simulink model "WBR_Simulator"  (R2023b)
settings: Solver=FixedStepAuto  StartTime=0.0  StopTime=60  FixedStep=0.001  MaxStep=0.001
undefined symbols (not defined in the file or in its folder): DiscIntNeverNeededParam, magnitude, robot_stats, SIMPARAM, X, Y, Z
libraries: sm_lib x73, nesl_utility x50, simulink x17, slpidlib x6, dsparch4 x2
(part 7 of 7)

== system WBR_Simulator/腿建模/并联腿1/运动学解算验证(仅可证明旋转矩阵 ==
  R : Inport
  R_inv : Inport  Port=2
  Bus Creator1 : BusCreator  Inputs=2
  Bus Creator3 : BusCreator  Inputs=2
  Discrete Derivative : simulink/Discrete/Discrete Derivative  gainval=1.0  ICPrevScaledInput=0.0  OutMin=[]  OutMax=[]  OutDataType=fixdt(1, 16)  OutScaling=2^-10  DoSatur=off
  Discrete Derivative1 : simulink/Discrete/Discrete Derivative  gainval=1.0  ICPrevScaledInput=0.0  OutMin=[]  OutMax=[]  OutDataType=fixdt(1, 16)  OutScaling=2^-10  DoSatur=off
  Mux : Mux  Inputs=2
  Mux1 : Mux  Inputs=2
  PS-Simulink Converter{4..7} (4 alike) : nesl_utility/PS-Simulink Converter  PhysicalDomain=network_engine_domain  SubClassName=ps_output  LeftPortType=input  RightPortType=output  PseudoPeriodic=off  Frequencies=[]  VectorFormat=1-D array  Unit=inherit  AffineConversion=off
  Product : Product
  Product1 : Product  Multiplication=Matrix(*)
  Product2 : Product  Multiplication=Matrix(*)
  Transform Sensor : sm_lib/Frames and Transforms/Transform Sensor  MeasurementFrame=Base  RotationSequence=XYX  SenseAngle=off  SenseAxis=off  SenseQ=off  SenseR=off  SenseRotationSequence=off  SenseOmegaX=off  SenseOmegaY=off  SenseOmegaZ=off  SenseOmega=off  SenseQDot=off  SenseRDot=off  SenseRotationSequenceDot=off  SenseAlphaX=off  SenseAlphaY=off  SenseAlphaZ=off  SenseAlpha=off  SenseQDDot=off  SenseRDDot=off  SenseX=on  SenseY=off  SenseZ=on  SenseXYZ=off  SenseRad=off  SenseAzim=off  SenseDist=off  SenseInc=off  SenseXDot=on  SenseYDot=off  SenseZDot=on  SenseXYZDot=off  SenseRadDot=off  SenseAzimDot=off  SenseDistDot=off  SenseIncDot=off  SenseXDDot=off  SenseYDDot=off  SenseZDDot=off  SenseXYZDDot=off  SenseRadDDot=off  SenseAzimDDot=off  SenseDistDDot=off  SenseIncDDot=off
  Zero-Order Hold{,1..3} (4 alike) : ZeroOrderHold  SampleTime=0.001
  笛卡尔转极坐标 : Subsystem
  五连杆末端坐标 : PMIOPort  Side=Right
  基坐标 : PMIOPort  Port=2  Side=Left
  wires:
  Discrete Derivative/1 -> Product/1
  Product1/1 -> ?  "代算C点正交坐标速度"
  [R] -> Product2/1
  Discrete Derivative1/1 -> Mux/2, Bus Creator1/2  "vd"
  笛卡尔转极坐标/2(L_0) -> Discrete Derivative1/1, Product/2
  Mux/1 -> Product1/2
  笛卡尔转极坐标/1(phi_0) -> Discrete Derivative/1
  [R_inv] -> Product1/1
  Product/1 -> Mux/1, Bus Creator1/1  "vq"
  PS-Simulink Converter5/1 -> Zero-Order Hold1/1
  Bus Creator1/1 -> ?  "真实C点极坐标速度"
  PS-Simulink Converter4/1 -> Zero-Order Hold/1
  Mux1/1 -> Product2/2
  Product2/1 -> ?  "代算C点极坐标速度"
  Bus Creator3/1 -> ?  "真实C点正交坐标速度"
  R/1 -> [R]
  R_inv/1 -> [R_inv]
  Zero-Order Hold/1 -> 笛卡尔转极坐标/1(x)
  Zero-Order Hold1/1 -> 笛卡尔转极坐标/2(z)
  Zero-Order Hold3/1 -> Mux1/2, Bus Creator3/2
  PS-Simulink Converter7/1 -> Zero-Order Hold3/1  "vz"
  Zero-Order Hold2/1 -> Mux1/1, Bus Creator3/1
  PS-Simulink Converter6/1 -> Zero-Order Hold2/1  "vx"
  connections:
  PS-Simulink Converter5/LConn1 -- Transform Sensor/RConn3
  PS-Simulink Converter4/LConn1 -- Transform Sensor/RConn2
  Transform Sensor/RConn1 -- 五连杆末端坐标/RConn1
  基坐标/RConn1 -- Transform Sensor/LConn1
  PS-Simulink Converter6/LConn1 -- Transform Sensor/RConn4
  PS-Simulink Converter7/LConn1 -- Transform Sensor/RConn5

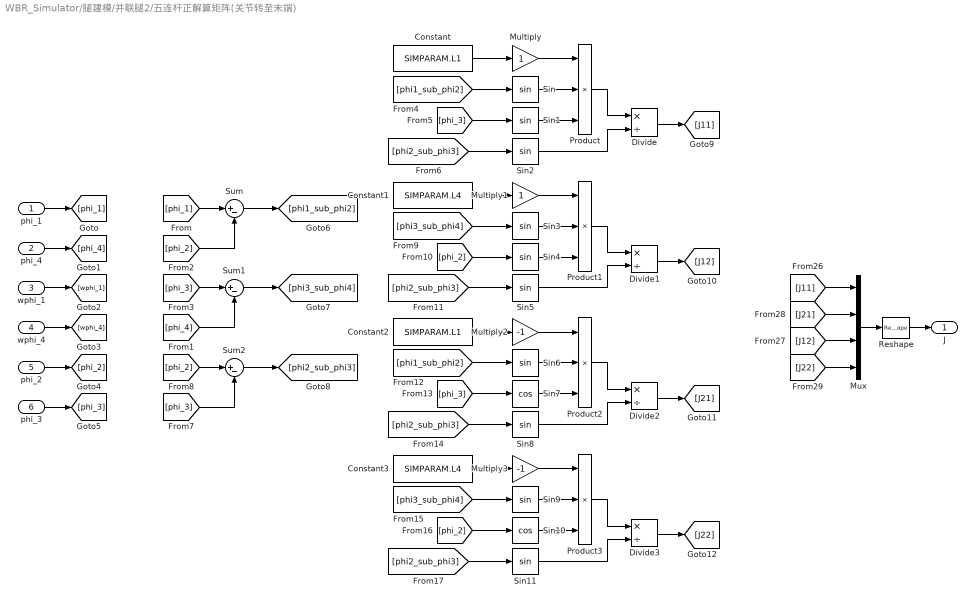
== system WBR_Simulator/腿建模/并联腿2/五连杆正解算矩阵(关节转至末端) ==
  phi_1 : Inport
  phi_4 : Inport  Port=2
  wphi_1 : Inport  Port=3
  wphi_4 : Inport  Port=4
  phi_2 : Inport  Port=5
  phi_3 : Inport  Port=6
  Constant : Constant  Value=SIMPARAM.L1
  Constant1 : Constant  Value=SIMPARAM.L4
  Constant2 : Constant  Value=SIMPARAM.L1
  Constant3 : Constant  Value=SIMPARAM.L4
  Divide{,1..3} (4 alike) : Product  Inputs=*/
  Multiply : Gain
  Multiply1 : Gain
  Multiply2 : Gain  Gain=-1
  Multiply3 : Gain  Gain=-1
  Mux : Mux
  Product{,1..3} (4 alike) : Product  Inputs=3
  Reshape : Reshape  OutputDimensionality=Customize  OutputDimensions=[2,2]
  Sin{,1..6,8..9,11} (10 alike) : Trigonometry
  Sin10 : Trigonometry  Operator=cos
  Sin7 : Trigonometry  Operator=cos
  Sum : Sum  Inputs=|+-
  Sum1 : Sum  Inputs=|+-
  Sum2 : Sum  Inputs=|+-
  J : Outport
  wires:
  phi_1/1 -> [phi_1]
  phi_4/1 -> [phi_4]
  wphi_1/1 -> [wphi_1]
  wphi_4/1 -> [wphi_4]
  phi_2/1 -> [phi_2]
  phi_3/1 -> [phi_3]
  [phi_1] -> Sum/1
  [phi_2] -> Sum/2
  Sum/1 -> [phi1_sub_phi2]
  Sum1/1 -> [phi3_sub_phi4]
  [phi_3] -> Sum1/1
  [phi_4] -> Sum1/2
  [phi1_sub_phi2] -> Sin/1
  Sin/1 -> Product/2
  Constant/1 -> Multiply/1
  Multiply/1 -> Product/1
  [phi_3] -> Sin1/1
  Sin1/1 -> Product/3
  Product/1 -> Divide/1
  [phi2_sub_phi3] -> Sin2/1
  Sin2/1 -> Divide/2
  [phi_3] -> Sum2/2
  [phi_2] -> Sum2/1
  Sum2/1 -> [phi2_sub_phi3]
  Divide/1 -> [J11]
  Product1/1 -> Divide1/1
  Constant1/1 -> Multiply1/1
  [phi3_sub_phi4] -> Sin3/1
  Divide1/1 -> [J12]
  Sin5/1 -> Divide1/2
  [phi_2] -> Sin4/1
  Multiply1/1 -> Product1/1
  Sin4/1 -> Product1/3
  [phi2_sub_phi3] -> Sin5/1
  Sin3/1 -> Product1/2
  Product2/1 -> Divide2/1
  Constant2/1 -> Multiply2/1
  [phi1_sub_phi2] -> Sin6/1
  Divide2/1 -> [J21]
  Sin8/1 -> Divide2/2
  [phi_3] -> Sin7/1
  Multiply2/1 -> Product2/1
  Sin7/1 -> Product2/3
  [phi2_sub_phi3] -> Sin8/1
  Sin6/1 -> Product2/2
  Product3/1 -> Divide3/1
  Constant3/1 -> Multiply3/1
  [phi3_sub_phi4] -> Sin9/1
  Divide3/1 -> [J22]
  Sin11/1 -> Divide3/2
  [phi_2] -> Sin10/1
  Multiply3/1 -> Product3/1
  Sin10/1 -> Product3/3
  [phi2_sub_phi3] -> Sin11/1
  Sin9/1 -> Product3/2
  [J11] -> Mux/1
  [J22] -> Mux/4
  Mux/1 -> Reshape/1
  Reshape/1 -> J/1
  [J21] -> Mux/2
  [J12] -> Mux/3

== system WBR_Simulator/腿建模/并联腿2/腿末端控制器 ==
  phi : Inport
  wphi_1 : Inport  Port=2
  wphi_4 : Inport  Port=3
  set_tq : Inport  Port=4
  set_fd : Inport  Port=5
  J : Inport  Port=6
  Bus Selector : BusSelector  OutputSignals=phi_1,phi_2
  Constant : Constant  Value=0
  Constant1 : Constant
  Constant2 : Constant
  Constant3 : Constant  Value=0
  Divide : Product  Inputs=*/
  Mux : Mux  Inputs=2
  Mux1 : Mux
  Product : Product  Inputs=/  Multiplication=Matrix(*)
  Product8 : Product  Multiplication=Matrix(*)
  Reshape : Reshape  OutputDimensionality=Customize  OutputDimensions=[2,2]
  极坐标运动控制器 : Subsystem
  笛卡尔坐标系转极坐标系 : Subsystem
  torque_1 : Outport
  torque_4 : Outport  Port=2
  R : Outport  Port=3
  R_inv : Outport  Port=4
  phi_0 : Outport  Port=5
  L_0 : Outport  Port=6
  real_vq : Outport  Port=7
  real_vd : Outport  Port=8
  valid_tqd : Outport  Port=9
  wires:
  J/1 -> [J]
  wphi_1/1 -> [wphi_1]
  wphi_4/1 -> [wphi_4]
  Product8/1 -> [real_vxy]
  [wphi_4] -> Mux/2
  [J] -> Product8/1
  Mux/1 -> Product8/2
  [wphi_1] -> Mux/1
  [real_vxy] -> 极坐标运动控制器/1(real_vxy)
  [R] -> 极坐标运动控制器/2(R)
  [J] -> 极坐标运动控制器/3(J)
  笛卡尔坐标系转极坐标系/1(R) -> [R], R/1, Product/1
  Product/1 -> R_inv/1
  极坐标运动控制器/2(torque_4) -> torque_4/1
  极坐标运动控制器/1(torque_1) -> torque_1/1
  笛卡尔坐标系转极坐标系/3(L_0) -> [L_0], L_0/1
  笛卡尔坐标系转极坐标系/2(phi_0) -> phi_0/1
  set_tq/1 -> 极坐标运动控制器/6(set_tq)
  set_fd/1 -> 极坐标运动控制器/7(set_fd)
  极坐标运动控制器/4(real_vd) -> real_vd/1
  极坐标运动控制器/3(real_vq) -> real_vq/1
  [phi_2] -> 笛卡尔坐标系转极坐标系/2(phi_2)
  [phi_1] -> 笛卡尔坐标系转极坐标系/1(phi_1)
  Mux1/1 -> Reshape/1
  [L_0] -> Divide/2
  Constant1/1 -> Mux1/4  "M22"
  Reshape/1 -> [M]
  [M] -> 极坐标运动控制器/4(M)
  Constant/1 -> Mux1/3  "M12"
  Constant3/1 -> Mux1/2  "M21"
  Constant2/1 -> Divide/1
  Divide/1 -> Mux1/1  "M11"
  极坐标运动控制器/5(valid_tqd) -> valid_tqd/1
  [phi] -> 极坐标运动控制器/5(In5)
  Bus Selector/1 -> [phi_1]  "<phi_1>"
  Bus Selector/2 -> [phi_2]  "<phi_2>"
  phi/1 -> [phi], Bus Selector/1

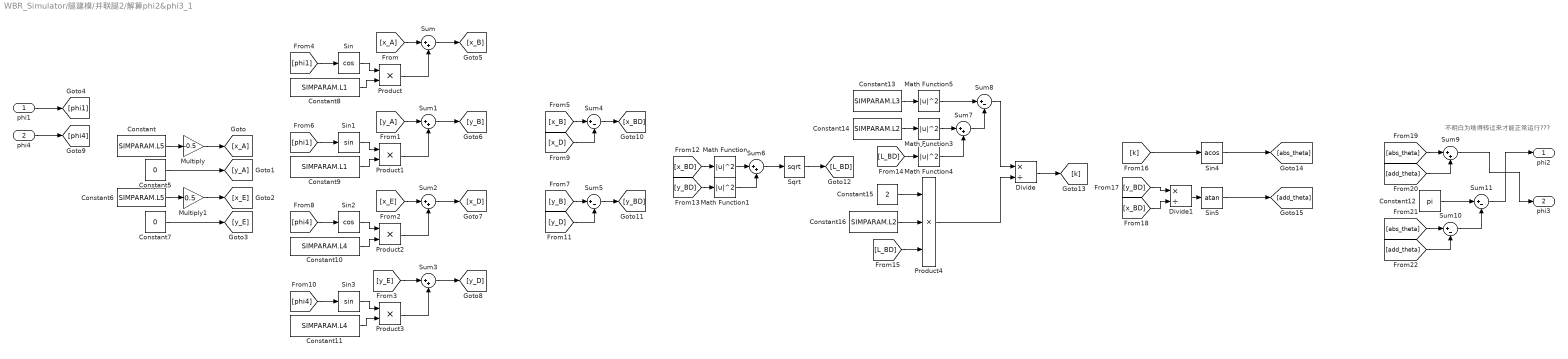
== system WBR_Simulator/腿建模/并联腿2/解算phi2&phi3_1 ==
  note: 不明白为啥得转过来才能正常运行???
  phi1 : Inport
  phi4 : Inport  Port=2
  Constant : Constant  Value=SIMPARAM.L5
  Constant10 : Constant  Value=SIMPARAM.L4
  Constant11 : Constant  Value=SIMPARAM.L4
  Constant12 : Constant  Value=pi
  Constant13 : Constant  Value=SIMPARAM.L3
  Constant14 : Constant  Value=SIMPARAM.L2
  Constant15 : Constant  Value=2
  Constant16 : Constant  Value=SIMPARAM.L2
  Constant5 : Constant  Value=0
  Constant6 : Constant  Value=SIMPARAM.L5
  Constant7 : Constant  Value=0
  Constant8 : Constant  Value=SIMPARAM.L1
  Constant9 : Constant  Value=SIMPARAM.L1
  Divide : Product  Inputs=*/
  Divide1 : Product  Inputs=*/
  Math Function{,1,3..5} (5 alike) : Math  Operator=magnitude^2
  Multiply : Gain  Gain=-0.5
  Multiply1 : Gain  Gain=0.5
  Product{,1..3} (4 alike) : Product
  Product4 : Product  Inputs=3
  Sin : Trigonometry  Operator=cos
  Sin1 : Trigonometry
  Sin2 : Trigonometry  Operator=cos
  Sin3 : Trigonometry
  Sin4 : Trigonometry  Operator=acos
  Sin5 : Trigonometry  Operator=atan
  Sqrt : Sqrt
  Sum{,1..3,6..7,9} (7 alike) : Sum  Inputs=|++
  Sum{4..5,8,10..11} (5 alike) : Sum  Inputs=|+-
  phi2 : Outport
  phi3 : Outport  Port=2
  wires:
  Constant/1 -> Multiply/1
  Multiply/1 -> [x_A]
  Constant5/1 -> [y_A]
  Multiply1/1 -> [x_E]
  Constant6/1 -> Multiply1/1
  Constant7/1 -> [y_E]
  [x_A] -> Sum/1
  [phi1] -> Sin/1
  Sin/1 -> Product/1
  Product/1 -> Sum/2
  Constant8/1 -> Product/2
  phi1/1 -> [phi1]
  Constant9/1 -> Product1/2
  Product1/1 -> Sum1/2
  Sin1/1 -> Product1/1
  [y_A] -> Sum1/1
  [phi1] -> Sin1/1
  Constant10/1 -> Product2/2
  Product2/1 -> Sum2/2
  Sin2/1 -> Product2/1
  [x_E] -> Sum2/1
  [phi4] -> Sin2/1
  Constant11/1 -> Product3/2
  Product3/1 -> Sum3/2
  Sin3/1 -> Product3/1
  [y_E] -> Sum3/1
  [phi4] -> Sin3/1
  Sum/1 -> [x_B]
  Sum1/1 -> [y_B]
  Sum2/1 -> [x_D]
  Sum3/1 -> [y_D]
  phi4/1 -> [phi4]
  [x_B] -> Sum4/1
  [x_D] -> Sum4/2
  [y_B] -> Sum5/1
  [y_D] -> Sum5/2
  Sum4/1 -> [x_BD]
  Sum5/1 -> [y_BD]
  [x_BD] -> Math Function/1
  [y_BD] -> Math Function1/1
  Math Function/1 -> Sum6/1
  Math Function1/1 -> Sum6/2
  Sum6/1 -> Sqrt/1
  Sqrt/1 -> [L_BD]
  Constant14/1 -> Math Function3/1
  [L_BD] -> Math Function4/1
  Sum7/1 -> Sum8/2
  Math Function3/1 -> Sum7/1
  Math Function4/1 -> Sum7/2
  Sum8/1 -> Divide/1
  [L_BD] -> Product4/3
  Constant15/1 -> Product4/1
  Constant16/1 -> Product4/2
  Product4/1 -> Divide/2
  Divide/1 -> [k]
  [k] -> Sin4/1
  [y_BD] -> Divide1/1
  Sin5/1 -> [add_theta]
  [abs_theta] -> Sum9/1
  [add_theta] -> Sum9/2
  [x_BD] -> Divide1/2
  [abs_theta] -> Sum10/1
  [add_theta] -> Sum10/2
  Constant13/1 -> Math Function5/1
  Math Function5/1 -> Sum8/1
  Sum10/1 -> Sum11/2
  Constant12/1 -> Sum11/1
  Sin4/1 -> [abs_theta]
  Divide1/1 -> Sin5/1
  Sum11/1 -> phi2/1
  Sum9/1 -> phi3/1

== system WBR_Simulator/腿建模/并联腿2/运动学解算验证(仅可证明旋转矩阵 ==
  R : Inport
  R_inv : Inport  Port=2
  Bus Creator1 : BusCreator  Inputs=2
  Bus Creator3 : BusCreator  Inputs=2
  Discrete Derivative : simulink/Discrete/Discrete Derivative  gainval=1.0  ICPrevScaledInput=0.0  OutMin=[]  OutMax=[]  OutDataType=fixdt(1, 16)  OutScaling=2^-10  DoSatur=off
  Discrete Derivative1 : simulink/Discrete/Discrete Derivative  gainval=1.0  ICPrevScaledInput=0.0  OutMin=[]  OutMax=[]  OutDataType=fixdt(1, 16)  OutScaling=2^-10  DoSatur=off
  Mux : Mux  Inputs=2
  Mux1 : Mux  Inputs=2
  PS-Simulink Converter{4..7} (4 alike) : nesl_utility/PS-Simulink Converter  PhysicalDomain=network_engine_domain  SubClassName=ps_output  LeftPortType=input  RightPortType=output  PseudoPeriodic=off  Frequencies=[]  VectorFormat=1-D array  Unit=inherit  AffineConversion=off
  Product : Product
  Product1 : Product  Multiplication=Matrix(*)
  Product2 : Product  Multiplication=Matrix(*)
  Transform Sensor : sm_lib/Frames and Transforms/Transform Sensor  MeasurementFrame=Base  RotationSequence=XYX  SenseAngle=off  SenseAxis=off  SenseQ=off  SenseR=off  SenseRotationSequence=off  SenseOmegaX=off  SenseOmegaY=off  SenseOmegaZ=off  SenseOmega=off  SenseQDot=off  SenseRDot=off  SenseRotationSequenceDot=off  SenseAlphaX=off  SenseAlphaY=off  SenseAlphaZ=off  SenseAlpha=off  SenseQDDot=off  SenseRDDot=off  SenseX=on  SenseY=off  SenseZ=on  SenseXYZ=off  SenseRad=off  SenseAzim=off  SenseDist=off  SenseInc=off  SenseXDot=on  SenseYDot=off  SenseZDot=on  SenseXYZDot=off  SenseRadDot=off  SenseAzimDot=off  SenseDistDot=off  SenseIncDot=off  SenseXDDot=off  SenseYDDot=off  SenseZDDot=off  SenseXYZDDot=off  SenseRadDDot=off  SenseAzimDDot=off  SenseDistDDot=off  SenseIncDDot=off
  Zero-Order Hold{,1..3} (4 alike) : ZeroOrderHold  SampleTime=0.001
  笛卡尔转极坐标 : Subsystem
  五连杆末端坐标 : PMIOPort  Side=Right
  基坐标 : PMIOPort  Port=2  Side=Left
  wires:
  Discrete Derivative/1 -> Product/1
  Product1/1 -> ?  "代算C点正交坐标速度"
  [R] -> Product2/1
  Discrete Derivative1/1 -> Mux/2, Bus Creator1/2  "vd"
  笛卡尔转极坐标/2(L_0) -> Discrete Derivative1/1, Product/2
  Mux/1 -> Product1/2
  笛卡尔转极坐标/1(phi_0) -> Discrete Derivative/1
  [R_inv] -> Product1/1
  Product/1 -> Mux/1, Bus Creator1/1  "vq"
  PS-Simulink Converter5/1 -> Zero-Order Hold1/1
  Bus Creator1/1 -> ?  "真实C点极坐标速度"
  PS-Simulink Converter4/1 -> Zero-Order Hold/1
  Mux1/1 -> Product2/2
  Product2/1 -> ?  "代算C点极坐标速度"
  Bus Creator3/1 -> ?  "真实C点正交坐标速度"
  R/1 -> [R]
  R_inv/1 -> [R_inv]
  Zero-Order Hold/1 -> 笛卡尔转极坐标/1(x)
  Zero-Order Hold1/1 -> 笛卡尔转极坐标/2(z)
  Zero-Order Hold3/1 -> Mux1/2, Bus Creator3/2
  PS-Simulink Converter7/1 -> Zero-Order Hold3/1  "vz"
  Zero-Order Hold2/1 -> Mux1/1, Bus Creator3/1
  PS-Simulink Converter6/1 -> Zero-Order Hold2/1  "vx"
  connections:
  PS-Simulink Converter5/LConn1 -- Transform Sensor/RConn3
  PS-Simulink Converter4/LConn1 -- Transform Sensor/RConn2
  Transform Sensor/RConn1 -- 五连杆末端坐标/RConn1
  基坐标/RConn1 -- Transform Sensor/LConn1
  PS-Simulink Converter6/LConn1 -- Transform Sensor/RConn4
  PS-Simulink Converter7/LConn1 -- Transform Sensor/RConn5

== system WBR_Simulator/腿建模/串联腿/腿末端控制器/xy运动 ==
  note: 参数对应无质量
  real_vxy : Inport
  J : Inport  Port=2
  Clock : Clock
  Clock1 : Clock
  Demux1 : Demux  Outputs=2
  Demux2 : Demux  Outputs=2
  Multiply2 : Gain  Gain=0.1
  Multiply3 : Gain  Gain=2*pi*1
  Multiply4 : Gain  Gain=0.1
  Multiply5 : Gain  Gain=5
  Multiply6 : Gain  Gain=5
  Multiply7 : Gain  Gain=2*pi*1
  Mux2 : Mux  Inputs=2
  Product10 : Product  Multiplication=Matrix(*)
  Product9 : Product  Inputs=/  Multiplication=Matrix(*)
  Sin : Trigonometry  Operator=cos
  Sin1 : Trigonometry
  Sum4 : Sum  Inputs=|+-
  Sum5 : Sum  Inputs=|+-
  Transpose1 : Math  Operator=transpose
  torque_1 : Outport
  torque_4 : Outport  Port=2
  wires:
  Multiply4/1 -> Sum4/1
  [real_vy] -> Sum5/2
  [real_vxy] -> Demux1/1
  Sum5/1 -> Multiply6/1
  Transpose1/1 -> Product9/1
  [real_vx] -> Sum4/2
  Multiply6/1 -> Mux2/2
  Clock1/1 -> Multiply7/1
  [J] -> Transpose1/1
  Multiply7/1 -> Sin1/1
  Demux2/1 -> torque_1/1
  Sin1/1 -> Multiply2/1
  Product10/1 -> Demux2/1
  Mux2/1 -> [set_txy]
  Multiply5/1 -> Mux2/1
  Product9/1 -> Product10/1
  Sin/1 -> Multiply4/1
  Demux2/2 -> torque_4/1
  Sum4/1 -> Multiply5/1
  Clock/1 -> Multiply3/1
  Multiply3/1 -> Sin/1
  [set_txy] -> Product10/2
  Demux1/1 -> [real_vx]
  Demux1/2 -> [real_vy]
  Multiply2/1 -> Sum5/1
  real_vxy/1 -> [real_vxy]
  J/1 -> [J]

== system WBR_Simulator/腿建模/串联腿/腿末端控制器/极坐标运动控制器 ==
  note: 解算实际姿态
  note: 解算控制力矩
  note: 获得Fx,Fy
  note: 获得Fq,Fd
  real_vxy : Inport
  R : Inport  Port=2
  J : Inport  Port=3
  M : Inport  Port=4
  In5 : Inport  Port=5
  set_tq : Inport  Port=6
  set_fd : Inport  Port=7
  Bus Selector : BusSelector  OutputSignals=phi_1,phi_2
  Demux : Demux  Outputs=2
  Demux2 : Demux  Outputs=2
  From : From  Commented=on  GotoTag=M
  From10 : From  Commented=on  GotoTag=R
  From11 : From  Commented=on  GotoTag=set_tqd
  From12 : From  Commented=on  GotoTag=J
  Matrix Multiply{,1..5} (6 alike) : Product  Multiplication=Matrix(*)
  Mux : Mux  Inputs=2
  Mux1 : Mux  Inputs=2
  Product{,2..3,5} (4 alike) : Product  Inputs=/  Multiplication=Matrix(*)
  Product1 : Product  Multiplication=Matrix(*)
  Product4 : Product  Commented=on  Inputs=4  Multiplication=Matrix(*)
  Saturation : Saturate  UpperLimit=robot_stats.max_torque_joint  LowerLimit=-robot_stats.max_torque_joint
  Saturation1 : Saturate  UpperLimit=robot_stats.max_torque_joint  LowerLimit=-robot_stats.max_torque_joint
  Transpose1 : Math  Commented=on  Operator=transpose
  Transpose2 : Math  Operator=transpose
  Transpose3 : Math  Operator=transpose
  torque_1 : Outport
  torque_2 : Outport  Port=2
  real_vq : Outport  Port=3
  real_vd : Outport  Port=4
  valid_tqd : Outport  Port=5
  wires:
  Demux/1 -> real_vq/1
  Product1/1 -> [real_vqd]
  From11/1 -> Product4/4
  R/1 -> [R]
  J/1 -> [J]
  From12/1 -> Transpose1/1
  Transpose1/1 -> Product4/1
  [R] -> Product5/1
  From10/1 -> Product4/2
  Demux/2 -> real_vd/1
  M/1 -> [M]
  From/1 -> Product4/3
  [M] -> Matrix Multiply/1
  [R] -> Matrix Multiply1/1
  [J] -> Transpose2/1
  Matrix Multiply2/1 -> Demux2/1
  Matrix Multiply/1 -> Matrix Multiply1/2
  Transpose2/1 -> Matrix Multiply2/1
  [real_vqd] -> Demux/1
  real_vxy/1 -> Product1/2
  Matrix Multiply1/1 -> Matrix Multiply2/2
  Mux/1 -> [real_t12]
  Saturation1/1 -> Mux/2, torque_2/1
  Saturation/1 -> Mux/1, torque_1/1
  [J] -> Transpose3/1
  Transpose3/1 -> Product/1
  Product/1 -> Matrix Multiply3/1
  [real_t12] -> Matrix Multiply3/2
  [R] -> Product2/1
  Product2/1 -> Matrix Multiply4/1
  Matrix Multiply3/1 -> Matrix Multiply4/2
  [M] -> Product3/1
  Product3/1 -> Matrix Multiply5/1
  Matrix Multiply4/1 -> Matrix Multiply5/2
  Matrix Multiply5/1 -> valid_tqd/1
  Demux2/2 -> Saturation1/1
  Demux2/1 -> Saturation/1
  In5/1 -> Bus Selector/1
  Bus Selector/1 -> [phi_1]  "<phi_1>"
  Bus Selector/2 -> [phi_2]  "<phi_2>"
  set_tq/1 -> Mux1/1
  set_fd/1 -> Mux1/2
  Mux1/1 -> Matrix Multiply/2
  Product5/1 -> Product1/1

== system WBR_Simulator/腿建模/串联腿/腿末端控制器/笛卡尔坐标系转极坐标系 ==
  note: 逆时针的Fq方为正
  phi_1 : Inport
  phi_2 : Inport  Port=2
  Constant : Constant  Value=pi/2
  Constant1 : Constant  Value=SIMPARAM.L2
  Constant5 : Constant  Value=SIMPARAM.L1
  Constant7 : Constant  Value=SIMPARAM.L2
  Constant8 : Constant  Value=SIMPARAM.L1
  Math Function : Math  Operator=magnitude^2
  Math Function1 : Math  Operator=magnitude^2
  Multiply1 : Gain  Gain=-1
  Mux : Mux
  Product{,1..3} (4 alike) : Product
  Reshape : Reshape  OutputDimensionality=Customize  OutputDimensions=[2,2]
  Sin{,1,5,8} (4 alike) : Trigonometry  Operator=cos
  Sin{2..3,6..7} (4 alike) : Trigonometry
  Sin4 : Trigonometry  Operator=atan2
  Sqrt : Sqrt
  Sum : Sum  Inputs=|++
  Sum1 : Sum  Inputs=|++
  Sum2 : Sum  Inputs=|+-
  Sum3 : Sum  Inputs=|++
  R : Outport
  phi_0 : Outport  Port=2
  L_0 : Outport  Port=3
  wires:
  Constant7/1 -> Product2/1
  [phi_2] -> Sin/1
  Sin1/1 -> Product1/2
  Constant5/1 -> Product1/1
  [y_C] -> Sin4/1
  Sin3/1 -> Product3/2
  [phi_1] -> Sin1/1
  [phi_1] -> Sin3/1
  Product3/1 -> Sum1/2
  [phi_2] -> Sin2/1
  Sin2/1 -> Product2/2
  Constant8/1 -> Product3/1
  [x_C] -> Sin4/2
  Constant1/1 -> Product/1
  Sin/1 -> Product/2
  Product2/1 -> Sum1/1
  Sin4/1 -> [phi_C]
  Sin5/1 -> [R21]
  Sin6/1 -> [R22]
  [R11] -> Mux/1  "R11"
  [R21] -> Mux/2  "R21"
  [R12] -> Mux/3  "R12"
  [R22] -> Mux/4  "R22"
  Mux/1 -> Reshape/1
  [y_C] -> Math Function/1
  [x_C] -> Math Function1/1
  Math Function/1 -> Sum3/1
  Math Function1/1 -> Sum3/2
  Sum3/1 -> Sqrt/1
  Sqrt/1 -> [L_0]
  [phi_C] -> Sin5/1
  [phi_C] -> Sin6/1
  [phi_C] -> Sum2/1
  phi_2/1 -> [phi_2]
  phi_1/1 -> [phi_1]
  Sum/1 -> [x_C]
  Sum1/1 -> [y_C]
  [L_0] -> L_0/1
  Sin7/1 -> Multiply1/1
  Multiply1/1 -> [R11]
  Sin8/1 -> [R12]
  [phi_C] -> Sin8/1
  Sum2/1 -> phi_0/1
  Reshape/1 -> R/1
  Constant/1 -> Sum2/2
  [phi_C] -> Sin7/1
  Product/1 -> Sum/1
  Product1/1 -> Sum/2

== system WBR_Simulator/腿建模/串联腿/运动学解算验证(仅可证明旋转矩阵/笛卡尔转极坐标 ==
  x : Inport
  z : Inport  Port=2
  Math Function : Math  Operator=magnitude^2
  Math Function1 : Math  Operator=magnitude^2
  Sin : Trigonometry  Operator=atan2
  Sqrt : Sqrt
  Sum : Sum  Inputs=|++
  phi_0 : Outport
  L_0 : Outport  Port=2
  wires:
  z/1 -> Math Function/1, Sin/1
  x/1 -> Sin/2, Math Function1/1
  Sin/1 -> phi_0/1
  Math Function/1 -> Sum/1
  Math Function1/1 -> Sum/2
  Sum/1 -> Sqrt/1
  Sqrt/1 -> L_0/1

== system WBR_Simulator/腿建模/并联腿/腿末端控制器/极坐标运动控制器 ==
  note: 解算实际姿态
  note: 解算控制力矩
  note: 获得Fx,Fy
  note: 获得Fq,Fd
  real_vxy : Inport
  R : Inport  Port=2
  J : Inport  Port=3
  M : Inport  Port=4
  In5 : Inport  Port=5
  set_tq : Inport  Port=6
  set_fd : Inport  Port=7
  Bus Selector : BusSelector  OutputSignals=phi_1,phi_2,phi_3,phi_4
  Demux : Demux  Outputs=2
  Demux2 : Demux  Outputs=2
  From : From  Commented=on  GotoTag=M
  From10 : From  Commented=on  GotoTag=R
  From11 : From  Commented=on  GotoTag=set_tqd
  From12 : From  Commented=on  GotoTag=J
  Matrix Multiply{,1..5} (6 alike) : Product  Multiplication=Matrix(*)
  Mux : Mux  Inputs=2
  Mux1 : Mux  Inputs=2
  Product : Product  Inputs=/  Multiplication=Matrix(*)
  Product1 : Product  Multiplication=Matrix(*)
  Product2 : Product  Inputs=/  Multiplication=Matrix(*)
  Product3 : Product  Inputs=/  Multiplication=Matrix(*)
  Product4 : Product  Commented=on  Inputs=4  Multiplication=Matrix(*)
  Saturation : Saturate  UpperLimit=robot_stats.max_torque_joint  LowerLimit=-robot_stats.max_torque_joint
  Saturation1 : Saturate  UpperLimit=robot_stats.max_torque_joint  LowerLimit=-robot_stats.max_torque_joint
  Transpose1 : Math  Commented=on  Operator=transpose
  Transpose2 : Math  Operator=transpose
  Transpose3 : Math  Operator=transpose
  torque_1 : Outport
  torque_4 : Outport  Port=2
  real_vq : Outport  Port=3
  real_vd : Outport  Port=4
  valid_tqd : Outport  Port=5
  wires:
  Demux/1 -> real_vq/1
  Product1/1 -> [real_vqd]
  From11/1 -> Product4/4
  R/1 -> [R]
  J/1 -> [J]
  From12/1 -> Transpose1/1
  Transpose1/1 -> Product4/1
  [R] -> Product1/1
  From10/1 -> Product4/2
  Demux/2 -> real_vd/1
  M/1 -> [M]
  From/1 -> Product4/3
  [M] -> Matrix Multiply/1
  [R] -> Matrix Multiply1/1
  [J] -> Transpose2/1
  Matrix Multiply2/1 -> Demux2/1
  Matrix Multiply/1 -> Matrix Multiply1/2
  Transpose2/1 -> Matrix Multiply2/1
  [real_vqd] -> Demux/1
  real_vxy/1 -> Product1/2
  Matrix Multiply1/1 -> Matrix Multiply2/2
  Mux/1 -> [real_t14]
  Saturation1/1 -> Mux/2, torque_4/1
  Saturation/1 -> Mux/1, torque_1/1
  [J] -> Transpose3/1
  Transpose3/1 -> Product/1
  Product/1 -> Matrix Multiply3/1
  [real_t14] -> Matrix Multiply3/2
  [R] -> Product2/1
  Product2/1 -> Matrix Multiply4/1
  Matrix Multiply3/1 -> Matrix Multiply4/2
  [M] -> Product3/1
  Product3/1 -> Matrix Multiply5/1
  Matrix Multiply4/1 -> Matrix Multiply5/2
  Matrix Multiply5/1 -> valid_tqd/1
  Demux2/2 -> Saturation1/1
  Demux2/1 -> Saturation/1
  In5/1 -> Bus Selector/1
  Bus Selector/1 -> [phi_1]  "<phi_1>"
  Bus Selector/2 -> [phi_2]  "<phi_2>"
  Bus Selector/4 -> [phi_4]  "<phi_4>"
  Bus Selector/3 -> [phi_3]  "<phi_3>"
  set_tq/1 -> Mux1/1
  set_fd/1 -> Mux1/2
  Mux1/1 -> Matrix Multiply/2

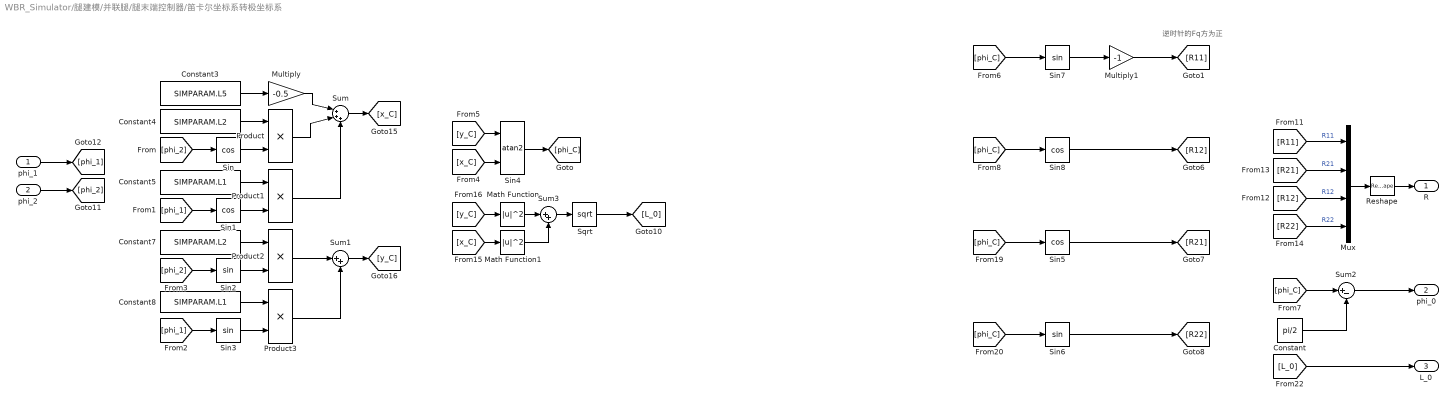
== system WBR_Simulator/腿建模/并联腿/腿末端控制器/笛卡尔坐标系转极坐标系 ==
  note: 逆时针的Fq方为正
  phi_1 : Inport
  phi_2 : Inport  Port=2
  Constant : Constant  Value=pi/2
  Constant3 : Constant  Value=SIMPARAM.L5
  Constant4 : Constant  Value=SIMPARAM.L2
  Constant5 : Constant  Value=SIMPARAM.L1
  Constant7 : Constant  Value=SIMPARAM.L2
  Constant8 : Constant  Value=SIMPARAM.L1
  Math Function : Math  Operator=magnitude^2
  Math Function1 : Math  Operator=magnitude^2
  Multiply : Gain  Gain=-0.5
  Multiply1 : Gain  Gain=-1
  Mux : Mux
  Product{,1..3} (4 alike) : Product
  Reshape : Reshape  OutputDimensionality=Customize  OutputDimensions=[2,2]
  Sin{,1,5,8} (4 alike) : Trigonometry  Operator=cos
  Sin{2..3,6..7} (4 alike) : Trigonometry
  Sin4 : Trigonometry  Operator=atan2
  Sqrt : Sqrt
  Sum : Sum  Inputs=|+++
  Sum1 : Sum  Inputs=|++
  Sum2 : Sum  Inputs=|+-
  Sum3 : Sum  Inputs=|++
  R : Outport
  phi_0 : Outport  Port=2
  L_0 : Outport  Port=3
  wires:
  Constant7/1 -> Product2/1
  Multiply/1 -> Sum/1
  Product1/1 -> Sum/3
  [phi_2] -> Sin/1
  Sin1/1 -> Product1/2
  Constant5/1 -> Product1/1
  [y_C] -> Sin4/1
  Sin3/1 -> Product3/2
  [phi_1] -> Sin1/1
  Constant3/1 -> Multiply/1
  [phi_1] -> Sin3/1
  Product3/1 -> Sum1/2
  [phi_2] -> Sin2/1
  Sin2/1 -> Product2/2
  Constant8/1 -> Product3/1
  [x_C] -> Sin4/2
  Constant4/1 -> Product/1
  Sin/1 -> Product/2
  Product/1 -> Sum/2
  Product2/1 -> Sum1/1
  Sin4/1 -> [phi_C]
  Sin5/1 -> [R21]
  Sin6/1 -> [R22]
  [R11] -> Mux/1  "R11"
  [R21] -> Mux/2  "R21"
  [R12] -> Mux/3  "R12"
  [R22] -> Mux/4  "R22"
  Mux/1 -> Reshape/1
  [y_C] -> Math Function/1
  [x_C] -> Math Function1/1
  Math Function/1 -> Sum3/1
  Math Function1/1 -> Sum3/2
  Sum3/1 -> Sqrt/1
  Sqrt/1 -> [L_0]
  [phi_C] -> Sin5/1
  [phi_C] -> Sin6/1
  [phi_C] -> Sum2/1
  phi_2/1 -> [phi_2]
  phi_1/1 -> [phi_1]
  Sum/1 -> [x_C]
  Sum1/1 -> [y_C]
  [L_0] -> L_0/1
  Sin7/1 -> Multiply1/1
  Multiply1/1 -> [R11]
  Sin8/1 -> [R12]
  [phi_C] -> Sin8/1
  Sum2/1 -> phi_0/1
  Reshape/1 -> R/1
  Constant/1 -> Sum2/2
  [phi_C] -> Sin7/1

== system WBR_Simulator/腿建模/并联腿/运动学解算验证(仅可证明旋转矩阵/笛卡尔转极坐标 ==
  x : Inport
  z : Inport  Port=2
  Math Function : Math  Operator=magnitude^2
  Math Function1 : Math  Operator=magnitude^2
  Sin : Trigonometry  Operator=atan2
  Sqrt : Sqrt
  Sum : Sum  Inputs=|++
  phi_0 : Outport
  L_0 : Outport  Port=2
  wires:
  z/1 -> Math Function/1, Sin/1
  x/1 -> Sin/2, Math Function1/1
  Sin/1 -> phi_0/1
  Math Function/1 -> Sum/1
  Math Function1/1 -> Sum/2
  Sum/1 -> Sqrt/1
  Sqrt/1 -> L_0/1

== system WBR_Simulator/腿建模/并联腿1/腿末端控制器/极坐标运动控制器 ==
  note: 解算实际姿态
  note: 解算控制力矩
  note: 获得Fx,Fy
  note: 获得Fq,Fd
  real_vxy : Inport
  R : Inport  Port=2
  J : Inport  Port=3
  M : Inport  Port=4
  In5 : Inport  Port=5
  set_tq : Inport  Port=6
  set_fd : Inport  Port=7
  Bus Selector : BusSelector  OutputSignals=phi_1,phi_2,phi_3,phi_4
  Demux : Demux  Outputs=2
  Demux2 : Demux  Outputs=2
  From : From  Commented=on  GotoTag=M
  From10 : From  Commented=on  GotoTag=R
  From11 : From  Commented=on  GotoTag=set_tqd
  From12 : From  Commented=on  GotoTag=J
  Matrix Multiply{,1..5} (6 alike) : Product  Multiplication=Matrix(*)
  Mux : Mux  Inputs=2
  Mux1 : Mux  Inputs=2
  Product : Product  Inputs=/  Multiplication=Matrix(*)
  Product1 : Product  Multiplication=Matrix(*)
  Product2 : Product  Inputs=/  Multiplication=Matrix(*)
  Product3 : Product  Inputs=/  Multiplication=Matrix(*)
  Product4 : Product  Commented=on  Inputs=4  Multiplication=Matrix(*)
  Saturation : Saturate  UpperLimit=robot_stats.max_torque_joint  LowerLimit=-robot_stats.max_torque_joint
  Saturation1 : Saturate  UpperLimit=robot_stats.max_torque_joint  LowerLimit=-robot_stats.max_torque_joint
  Transpose1 : Math  Commented=on  Operator=transpose
  Transpose2 : Math  Operator=transpose
  Transpose3 : Math  Operator=transpose
  torque_1 : Outport
  torque_4 : Outport  Port=2
  real_vq : Outport  Port=3
  real_vd : Outport  Port=4
  valid_tqd : Outport  Port=5
  wires:
  Demux/1 -> real_vq/1
  Product1/1 -> [real_vqd]
  From11/1 -> Product4/4
  R/1 -> [R]
  J/1 -> [J]
  From12/1 -> Transpose1/1
  Transpose1/1 -> Product4/1
  [R] -> Product1/1
  From10/1 -> Product4/2
  Demux/2 -> real_vd/1
  M/1 -> [M]
  From/1 -> Product4/3
  [M] -> Matrix Multiply/1
  [R] -> Matrix Multiply1/1
  [J] -> Transpose2/1
  Matrix Multiply2/1 -> Demux2/1
  Matrix Multiply/1 -> Matrix Multiply1/2
  Transpose2/1 -> Matrix Multiply2/1
  [real_vqd] -> Demux/1
  real_vxy/1 -> Product1/2
  Matrix Multiply1/1 -> Matrix Multiply2/2
  Mux/1 -> [real_t14]
  Saturation1/1 -> Mux/2, torque_4/1
  Saturation/1 -> Mux/1, torque_1/1
  [J] -> Transpose3/1
  Transpose3/1 -> Product/1
  Product/1 -> Matrix Multiply3/1
  [real_t14] -> Matrix Multiply3/2
  [R] -> Product2/1
  Product2/1 -> Matrix Multiply4/1
  Matrix Multiply3/1 -> Matrix Multiply4/2
  [M] -> Product3/1
  Product3/1 -> Matrix Multiply5/1
  Matrix Multiply4/1 -> Matrix Multiply5/2
  Matrix Multiply5/1 -> valid_tqd/1
  Demux2/2 -> Saturation1/1
  Demux2/1 -> Saturation/1
  In5/1 -> Bus Selector/1
  Bus Selector/1 -> [phi_1]  "<phi_1>"
  Bus Selector/2 -> [phi_2]  "<phi_2>"
  Bus Selector/4 -> [phi_4]  "<phi_4>"
  Bus Selector/3 -> [phi_3]  "<phi_3>"
  set_tq/1 -> Mux1/1
  set_fd/1 -> Mux1/2
  Mux1/1 -> Matrix Multiply/2

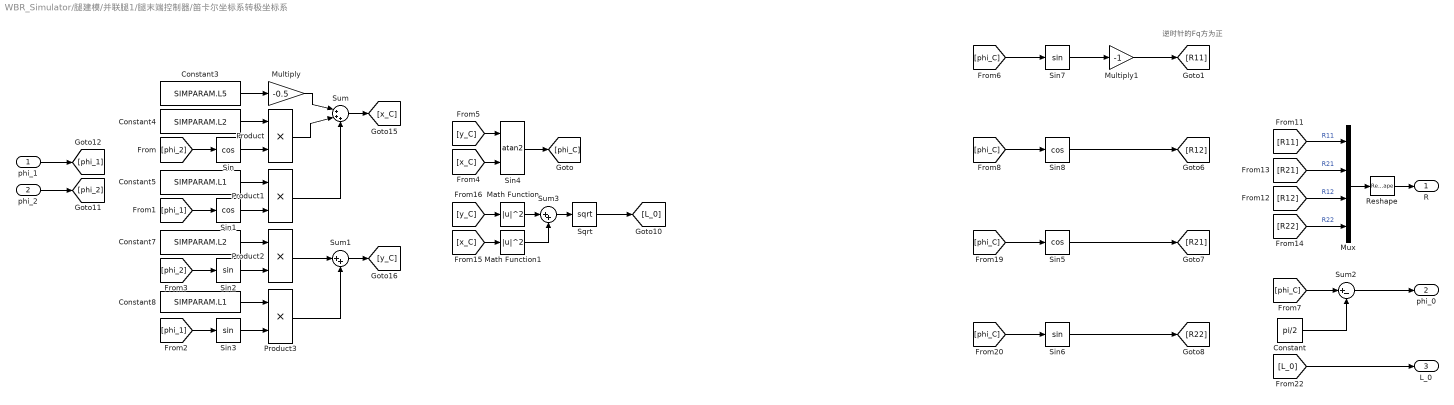
== system WBR_Simulator/腿建模/并联腿1/腿末端控制器/笛卡尔坐标系转极坐标系 ==
  note: 逆时针的Fq方为正
  phi_1 : Inport
  phi_2 : Inport  Port=2
  Constant : Constant  Value=pi/2
  Constant3 : Constant  Value=SIMPARAM.L5
  Constant4 : Constant  Value=SIMPARAM.L2
  Constant5 : Constant  Value=SIMPARAM.L1
  Constant7 : Constant  Value=SIMPARAM.L2
  Constant8 : Constant  Value=SIMPARAM.L1
  Math Function : Math  Operator=magnitude^2
  Math Function1 : Math  Operator=magnitude^2
  Multiply : Gain  Gain=-0.5
  Multiply1 : Gain  Gain=-1
  Mux : Mux
  Product{,1..3} (4 alike) : Product
  Reshape : Reshape  OutputDimensionality=Customize  OutputDimensions=[2,2]
  Sin{,1,5,8} (4 alike) : Trigonometry  Operator=cos
  Sin{2..3,6..7} (4 alike) : Trigonometry
  Sin4 : Trigonometry  Operator=atan2
  Sqrt : Sqrt
  Sum : Sum  Inputs=|+++
  Sum1 : Sum  Inputs=|++
  Sum2 : Sum  Inputs=|+-
  Sum3 : Sum  Inputs=|++
  R : Outport
  phi_0 : Outport  Port=2
  L_0 : Outport  Port=3
  wires:
  Constant7/1 -> Product2/1
  Multiply/1 -> Sum/1
  Product1/1 -> Sum/3
  [phi_2] -> Sin/1
  Sin1/1 -> Product1/2
  Constant5/1 -> Product1/1
  [y_C] -> Sin4/1
  Sin3/1 -> Product3/2
  [phi_1] -> Sin1/1
  Constant3/1 -> Multiply/1
  [phi_1] -> Sin3/1
  Product3/1 -> Sum1/2
  [phi_2] -> Sin2/1
  Sin2/1 -> Product2/2
  Constant8/1 -> Product3/1
  [x_C] -> Sin4/2
  Constant4/1 -> Product/1
  Sin/1 -> Product/2
  Product/1 -> Sum/2
  Product2/1 -> Sum1/1
  Sin4/1 -> [phi_C]
  Sin5/1 -> [R21]
  Sin6/1 -> [R22]
  [R11] -> Mux/1  "R11"
  [R21] -> Mux/2  "R21"
  [R12] -> Mux/3  "R12"
  [R22] -> Mux/4  "R22"
  Mux/1 -> Reshape/1
  [y_C] -> Math Function/1
  [x_C] -> Math Function1/1
  Math Function/1 -> Sum3/1
  Math Function1/1 -> Sum3/2
  Sum3/1 -> Sqrt/1
  Sqrt/1 -> [L_0]
  [phi_C] -> Sin5/1
  [phi_C] -> Sin6/1
  [phi_C] -> Sum2/1
  phi_2/1 -> [phi_2]
  phi_1/1 -> [phi_1]
  Sum/1 -> [x_C]
  Sum1/1 -> [y_C]
  [L_0] -> L_0/1
  Sin7/1 -> Multiply1/1
  Multiply1/1 -> [R11]
  Sin8/1 -> [R12]
  [phi_C] -> Sin8/1
  Sum2/1 -> phi_0/1
  Reshape/1 -> R/1
  Constant/1 -> Sum2/2
  [phi_C] -> Sin7/1

== system WBR_Simulator/腿建模/并联腿1/运动学解算验证(仅可证明旋转矩阵/笛卡尔转极坐标 ==
  x : Inport
  z : Inport  Port=2
  Math Function : Math  Operator=magnitude^2
  Math Function1 : Math  Operator=magnitude^2
  Sin : Trigonometry  Operator=atan2
  Sqrt : Sqrt
  Sum : Sum  Inputs=|++
  phi_0 : Outport
  L_0 : Outport  Port=2
  wires:
  z/1 -> Math Function/1, Sin/1
  x/1 -> Sin/2, Math Function1/1
  Sin/1 -> phi_0/1
  Math Function/1 -> Sum/1
  Math Function1/1 -> Sum/2
  Sum/1 -> Sqrt/1
  Sqrt/1 -> L_0/1

== system WBR_Simulator/腿建模/并联腿2/腿末端控制器/极坐标运动控制器 ==
  note: 解算实际姿态
  note: 解算控制力矩
  note: 获得Fx,Fy
  note: 获得Fq,Fd
  real_vxy : Inport
  R : Inport  Port=2
  J : Inport  Port=3
  M : Inport  Port=4
  In5 : Inport  Port=5
  set_tq : Inport  Port=6
  set_fd : Inport  Port=7
  Bus Selector : BusSelector  OutputSignals=phi_1,phi_2,phi_3,phi_4
  Demux : Demux  Outputs=2
  Demux2 : Demux  Outputs=2
  From : From  Commented=on  GotoTag=M
  From10 : From  Commented=on  GotoTag=R
  From11 : From  Commented=on  GotoTag=set_tqd
  From12 : From  Commented=on  GotoTag=J
  Matrix Multiply{,1..5} (6 alike) : Product  Multiplication=Matrix(*)
  Mux : Mux  Inputs=2
  Mux1 : Mux  Inputs=2
  Product : Product  Inputs=/  Multiplication=Matrix(*)
  Product1 : Product  Multiplication=Matrix(*)
  Product2 : Product  Inputs=/  Multiplication=Matrix(*)
  Product3 : Product  Inputs=/  Multiplication=Matrix(*)
  Product4 : Product  Commented=on  Inputs=4  Multiplication=Matrix(*)
  Saturation : Saturate  UpperLimit=robot_stats.max_torque_joint  LowerLimit=-robot_stats.max_torque_joint
  Saturation1 : Saturate  UpperLimit=robot_stats.max_torque_joint  LowerLimit=-robot_stats.max_torque_joint
  Transpose1 : Math  Commented=on  Operator=transpose
  Transpose2 : Math  Operator=transpose
  Transpose3 : Math  Operator=transpose
  torque_1 : Outport
  torque_4 : Outport  Port=2
  real_vq : Outport  Port=3
  real_vd : Outport  Port=4
  valid_tqd : Outport  Port=5
  wires:
  Demux/1 -> real_vq/1
  Product1/1 -> [real_vqd]
  From11/1 -> Product4/4
  R/1 -> [R]
  J/1 -> [J]
  From12/1 -> Transpose1/1
  Transpose1/1 -> Product4/1
  [R] -> Product1/1
  From10/1 -> Product4/2
  Demux/2 -> real_vd/1
  M/1 -> [M]
  From/1 -> Product4/3
  [M] -> Matrix Multiply/1
  [R] -> Matrix Multiply1/1
  [J] -> Transpose2/1
  Matrix Multiply2/1 -> Demux2/1
  Matrix Multiply/1 -> Matrix Multiply1/2
  Transpose2/1 -> Matrix Multiply2/1
  [real_vqd] -> Demux/1
  real_vxy/1 -> Product1/2
  Matrix Multiply1/1 -> Matrix Multiply2/2
  Mux/1 -> [real_t14]
  Saturation1/1 -> Mux/2, torque_4/1
  Saturation/1 -> Mux/1, torque_1/1
  [J] -> Transpose3/1
  Transpose3/1 -> Product/1
  Product/1 -> Matrix Multiply3/1
  [real_t14] -> Matrix Multiply3/2
  [R] -> Product2/1
  Product2/1 -> Matrix Multiply4/1
  Matrix Multiply3/1 -> Matrix Multiply4/2
  [M] -> Product3/1
  Product3/1 -> Matrix Multiply5/1
  Matrix Multiply4/1 -> Matrix Multiply5/2
  Matrix Multiply5/1 -> valid_tqd/1
  Demux2/2 -> Saturation1/1
  Demux2/1 -> Saturation/1
  In5/1 -> Bus Selector/1
  Bus Selector/1 -> [phi_1]  "<phi_1>"
  Bus Selector/2 -> [phi_2]  "<phi_2>"
  Bus Selector/4 -> [phi_4]  "<phi_4>"
  Bus Selector/3 -> [phi_3]  "<phi_3>"
  set_tq/1 -> Mux1/1
  set_fd/1 -> Mux1/2
  Mux1/1 -> Matrix Multiply/2

== system WBR_Simulator/腿建模/并联腿2/腿末端控制器/笛卡尔坐标系转极坐标系 ==
  note: 逆时针的Fq方为正
  phi_1 : Inport
  phi_2 : Inport  Port=2
  Constant : Constant  Value=pi/2
  Constant3 : Constant  Value=SIMPARAM.L5
  Constant4 : Constant  Value=SIMPARAM.L2
  Constant5 : Constant  Value=SIMPARAM.L1
  Constant7 : Constant  Value=SIMPARAM.L2
  Constant8 : Constant  Value=SIMPARAM.L1
  Math Function : Math  Operator=magnitude^2
  Math Function1 : Math  Operator=magnitude^2
  Multiply : Gain  Gain=-0.5
  Multiply1 : Gain  Gain=-1
  Mux : Mux
  Product{,1..3} (4 alike) : Product
  Reshape : Reshape  OutputDimensionality=Customize  OutputDimensions=[2,2]
  Sin{,1,5,8} (4 alike) : Trigonometry  Operator=cos
  Sin{2..3,6..7} (4 alike) : Trigonometry
  Sin4 : Trigonometry  Operator=atan2
  Sqrt : Sqrt
  Sum : Sum  Inputs=|+++
  Sum1 : Sum  Inputs=|++
  Sum2 : Sum  Inputs=|+-
  Sum3 : Sum  Inputs=|++
  R : Outport
  phi_0 : Outport  Port=2
  L_0 : Outport  Port=3
  wires:
  Constant7/1 -> Product2/1
  Multiply/1 -> Sum/1
  Product1/1 -> Sum/3
  [phi_2] -> Sin/1
  Sin1/1 -> Product1/2
  Constant5/1 -> Product1/1
  [y_C] -> Sin4/1
  Sin3/1 -> Product3/2
  [phi_1] -> Sin1/1
  Constant3/1 -> Multiply/1
  [phi_1] -> Sin3/1
  Product3/1 -> Sum1/2
  [phi_2] -> Sin2/1
  Sin2/1 -> Product2/2
  Constant8/1 -> Product3/1
  [x_C] -> Sin4/2
  Constant4/1 -> Product/1
  Sin/1 -> Product/2
  Product/1 -> Sum/2
  Product2/1 -> Sum1/1
  Sin4/1 -> [phi_C]
  Sin5/1 -> [R21]
  Sin6/1 -> [R22]
  [R11] -> Mux/1  "R11"
  [R21] -> Mux/2  "R21"
  [R12] -> Mux/3  "R12"
  [R22] -> Mux/4  "R22"
  Mux/1 -> Reshape/1
  [y_C] -> Math Function/1
  [x_C] -> Math Function1/1
  Math Function/1 -> Sum3/1
  Math Function1/1 -> Sum3/2
  Sum3/1 -> Sqrt/1
  Sqrt/1 -> [L_0]
  [phi_C] -> Sin5/1
  [phi_C] -> Sin6/1
  [phi_C] -> Sum2/1
  phi_2/1 -> [phi_2]
  phi_1/1 -> [phi_1]
  Sum/1 -> [x_C]
  Sum1/1 -> [y_C]
  [L_0] -> L_0/1
  Sin7/1 -> Multiply1/1
  Multiply1/1 -> [R11]
  Sin8/1 -> [R12]
  [phi_C] -> Sin8/1
  Sum2/1 -> phi_0/1
  Reshape/1 -> R/1
  Constant/1 -> Sum2/2
  [phi_C] -> Sin7/1

== system WBR_Simulator/腿建模/并联腿2/运动学解算验证(仅可证明旋转矩阵/笛卡尔转极坐标 ==
  x : Inport
  z : Inport  Port=2
  Math Function : Math  Operator=magnitude^2
  Math Function1 : Math  Operator=magnitude^2
  Sin : Trigonometry  Operator=atan2
  Sqrt : Sqrt
  Sum : Sum  Inputs=|++
  phi_0 : Outport
  L_0 : Outport  Port=2
  wires:
  z/1 -> Math Function/1, Sin/1
  x/1 -> Sin/2, Math Function1/1
  Sin/1 -> phi_0/1
  Math Function/1 -> Sum/1
  Math Function1/1 -> Sum/2
  Sum/1 -> Sqrt/1
  Sqrt/1 -> L_0/1

== matlab function WBR_Simulator/底盘控制器/MATLAB Function6 ==
  data: L_F_N input; flag output; R_F_N input; m input; g input
function flag = is_F_N_flag(L_F_N,R_F_N,m,g)
if L_F_N < m*g && R_F_N < m*g
    flag = 1;
else
    flag = 0;
end

== matlab function WBR_Simulator/腿建模/串联腿/五连杆正解算矩阵(关节转至末端)/MATLAB Function ==
  data: J11 input; J output; J12 input; J21 input; J22 input
function J = generateJ(J11,J12,J21,J22)

J = [
    J11,J12;
    J21,J22
];

== matlab function WBR_Simulator/底盘IMU/MATLAB Function1 ==
  data: quat_theta input; pitch output; yaw output; roll output
function [pitch,yaw,roll] = get_imu_data(quat_theta)
    quaternion=[quat_theta(1),quat_theta(2),quat_theta(3),quat_theta(4)];
 
    % 将四元数转换为旋转矩阵
    R  = quat2rotm(quaternion);   
    
    % 从旋转矩阵中提取所需的夹角
    % 计算相对于世界坐标系的 Z 轴夹角（yaw）
    yaw = atan2(R(2, 1), R(1, 1));
    
    % 求pitch
    % c0:imu系
    % c1:与车身同yaw但水平的坐标系
    % c2:车身坐标系
    R01 = [ cos(yaw) -sin(yaw) 0;
            sin(yaw) cos(yaw)  0;
            0        0         1];
    R02 = R;
    R12 = R01'* R02;

    % 计算 pitch 角
    %pitch = acos(R12(3,3))*sign(R12(3,1));
    pitch = atan2(R12(3,1), sqrt(R12(3,2)^2 + R12(3,3)^2));
    pitch = -pitch;

    % 计算 roll 角
    roll = atan2(R12(2, 3), R12(3, 3));
end

== matlab function WBR_Simulator/底盘控制器/限幅 ==
  data: T_w_lf input; T_w_rg input; T_p_lf input; T_p_rg input; Tx_l output; max_torque input; max_rpm input; real_vx_l input; Tx_r output; Tq_l output; Tq_r output; real_vx_r input
function [Tx_l,Tx_r,Tq_l,Tq_r]= wheel_controller(...
    T_w_lf,T_w_rg,...
    T_p_lf,T_p_rg,...
    max_torque,max_rpm,real_vx_l,real_vx_r)

    real_rpm_l=real_vx_l*30/pi;
    real_rpm_r=real_vx_r*30/pi;
    left_wheel_motor_torque=max_torque*(1-real_rpm_l/max_rpm);  
    right_wheel_motor_torque=max_torque*(1-real_rpm_l/max_rpm);  
    T_w_lf=clamp(T_w_lf,left_wheel_motor_torque);
    T_w_rg=clamp(T_w_rg,right_wheel_motor_torque);
    % Tqc=clamp(Tqc,20);
    % Tqd=clamp(Tqd,20);
    
    Tx_l = T_w_lf;
    Tx_r = T_w_rg;
    Tq_l = T_p_lf;
    Tq_r = T_p_rg;
end

function x=clamp(x,max)
    
     if (x>=0 && x>max)
       x=max;     
     end
     if (x<0 && x<-max)
       x=-max;
     end
end

== matlab function WBR_Simulator/底盘控制器/左腿离地检测1/MATLAB Function ==
  data: pitch input; az output; roll input; ax input; ay input; raw_az input
function az = calc_real_z(pitch, roll, ax, ay, raw_az)
sp = sin(pitch);
cp = cos(pitch);
sr = sin(roll);
cr = cos(roll);
az = -sp * ax + cp * sr * ay + cp * cr * raw_az;

== matlab function WBR_Simulator/底盘控制器/MATLAB Function2 ==
  data: K_LQR_param input; flag input; K_LQR output; L_l input; L_r input
function K_LQR = fcn(K_LQR_param,flag,L_l, L_r)
[i1,j1,k1,l1]=size(K_LQR_param);
K_LQR=zeros(i1,j1);
fn_k=zeros(i1,j1);
if flag == 1
    fn_k(3,5) = 1;
    fn_k(3,6) = 1;
    fn_k(3,7) = 1;
    fn_k(3,8) = 1;
    fn_k(4,5) = 1;
    fn_k(4,6) = 1;
    fn_k(4,7) = 1;
    fn_k(4,8) = 1;
else
    fn_k = ones(i1,j1);
end
% fn_k = ones(i1,j1);
for i=1:i1
    for j=1:j1
        for k=1:k1
            for l=1:l1
                K_LQR(i,j) = fn_k(i,j)*(K_LQR(i,j)+ K_LQR_param(i,j,k,l)*L_l^(k-1)*L_r^(l-1));
            end
        end
    end
end

== matlab function WBR_Simulator/底盘控制器/左腿离地检测2/MATLAB Function ==
  data: pitch input; az output; roll input; ax input; ay input; raw_az input
function az = calc_real_z(pitch, roll, ax, ay, raw_az)
sp = sin(pitch);
cp = cos(pitch);
sr = sin(roll);
cr = cos(roll);
az = -sp * ax + cp * sr * ay + cp * cr * raw_az;

== matlab function WBR_Simulator/底盘控制器/MATLAB Function4 ==
  data: exp_dx input; y output; cur_x input
function y = stop_flag(exp_dx,cur_x)
if(exp_dx ~= 0)
    cur_x = 0;
end
y = cur_x;

== matlab function WBR_Simulator/底盘控制器/MATLAB Function5 ==
  data: exp_dx input; dx output; cur_dx input; acc_max input
function dx = ddx_limit(exp_dx, cur_dx, acc_max)
dxmin = cur_dx - acc_max;
dxmax = cur_dx + acc_max;
limit_dx = exp_dx;
if exp_dx < dxmin
    limit_dx = dxmin;
end
if exp_dx > dxmax
    limit_dx = dxmax;
end
dx = limit_dx;
